simulink model "PerformanceMonitor"  (R2025b)
settings: Solver=VariableStepAuto  StartTime=0.0  StopTime=10.0  RelTol=1e-3
settings Model: Creator=Ishwar  LastModifiedBy=Ishwar

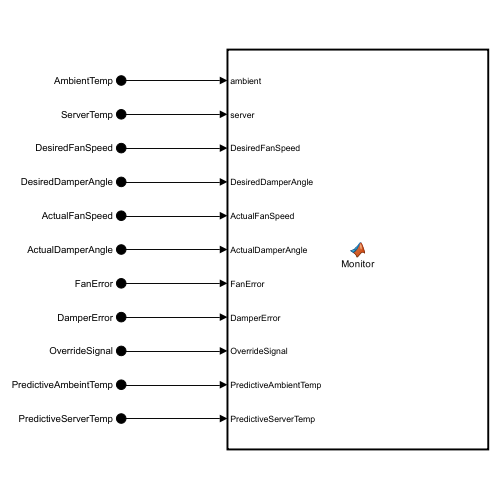
[thumbnail: Simulink's stored preview of the top-level diagram]
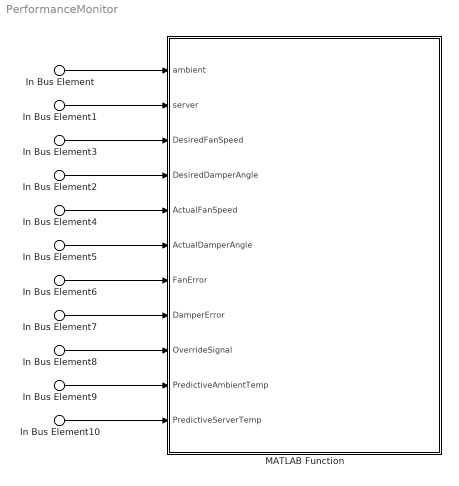
== system PerformanceMonitor ==
  In Bus Element : Inport  PortName=AmbientTemp
  In Bus Element1 : Inport  Port=2  PortName=ServerTemp
  In Bus Element2 : Inport  Port=3  PortName=DesiredDamperAngle
  In Bus Element3 : Inport  Port=4  PortName=DesiredFanSpeed
  In Bus Element4 : Inport  Port=5  PortName=ActualFanSpeed
  In Bus Element5 : Inport  Port=6  PortName=ActualDamperAngle
  In Bus Element6 : Inport  Port=7  PortName=FanError
  In Bus Element7 : Inport  Port=8  PortName=DamperError
  In Bus Element8 : Inport  Port=9  PortName=OverrideSignal
  In Bus Element9 : Inport  Port=10  PortName=PredictiveAmbeintTemp
  In Bus Element10 : Inport  Port=11  PortName=PredictiveServerTemp
  MATLAB Function : MATLAB Function  TreatAsAtomicUnit=on
  wires:
  In Bus Element8/1 -> MATLAB Function/9(OverrideSignal)
  In Bus Element7/1 -> MATLAB Function/8(DamperError)
  In Bus Element6/1 -> MATLAB Function/7(FanError)
  In Bus Element5/1 -> MATLAB Function/6(ActualDamperAngle)
  In Bus Element4/1 -> MATLAB Function/5(ActualFanSpeed)
  In Bus Element2/1 -> MATLAB Function/4(DesiredDamperAngle)
  In Bus Element3/1 -> MATLAB Function/3(DesiredFanSpeed)
  In Bus Element1/1 -> MATLAB Function/2(server)
  In Bus Element/1 -> MATLAB Function/1(ambient)
  In Bus Element9/1 -> MATLAB Function/10(PredictiveAmbientTemp)
  In Bus Element10/1 -> MATLAB Function/11(PredictiveServerTemp)

== matlab function PerformanceMonitor/MATLAB Function ==
  data: ambient input; server input; DesiredFanSpeed input; DesiredDamperAngle input; ActualFanSpeed input; ActualDamperAngle input; FanError input; DamperError input; OverrideSignal input; PredictiveAmbientTemp input; PredictiveServerTemp input
function Monitor(ambient, server, DesiredFanSpeed, DesiredDamperAngle, ActualFanSpeed, ActualDamperAngle, FanError, DamperError, OverrideSignal, PredictiveAmbientTemp, PredictiveServerTemp)
%#codegen

% Display sensor values
fprintf('--- Monitor Report ---\n');
fprintf('Ambient Temp: %.1f °C\n', ambient);
fprintf('Server Temp: %.1f °C\n', server);

% Display predictive values
fprintf('Predictive Ambient Temp: %.1f °C\n', PredictiveAmbientTemp);
fprintf('Predictive Server Temp: %.1f °C\n', PredictiveServerTemp);

% Display controller outputs
fprintf('Desired Fan Speed: %.1f %% (%.0f RPM)\n', DesiredFanSpeed, DesiredFanSpeed*100);
fprintf('Desired Damper Angle: %.1f °\n', DesiredDamperAngle);

% Display actuator outputs
fprintf('Actual Fan Speed: %.1f %% (%.0f RPM)\n', ActualFanSpeed, ActualFanSpeed*100);
fprintf('Actual Damper Angle: %.1f °\n', ActualDamperAngle);

% Display error feedback
fprintf('Fan Error: %.1f %% (%.0f RPM)\n', FanError, FanError*100);
fprintf('Damper Error: %.1f °\n', DamperError);

% Display override signal (cast to int for codegen safety)
fprintf('Override Signal: %d\n', int32(OverrideSignal));

% Alert if override triggered
if OverrideSignal ~= 0
    fprintf('*** ALERT: Override triggered due to error thresholds! ***\n');
end

fprintf('----------------------\n\n');
end
